simulink model "model_NLMPC_LMPCyawVar"  (R2024b)
settings: Solver=VariableStepAuto  StartTime=0.0  StopTime=25  RelTol=1e-3
undefined symbols (not defined in the file): drone, environment, traj
libraries: sharedtransform x2, mpclib x2, uavutilslib x1
settings Model: Creator=domac  LastModifiedBy=domac

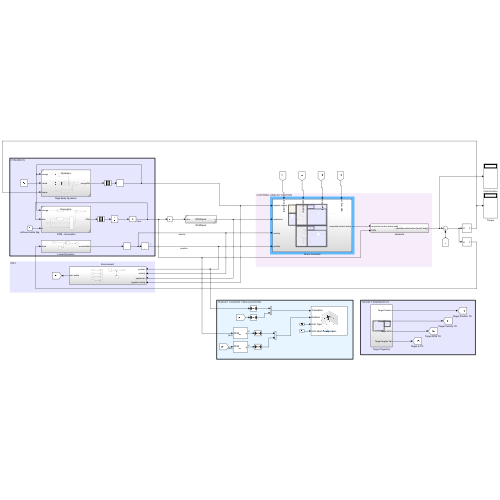
[thumbnail: Simulink's stored preview of the top-level diagram]
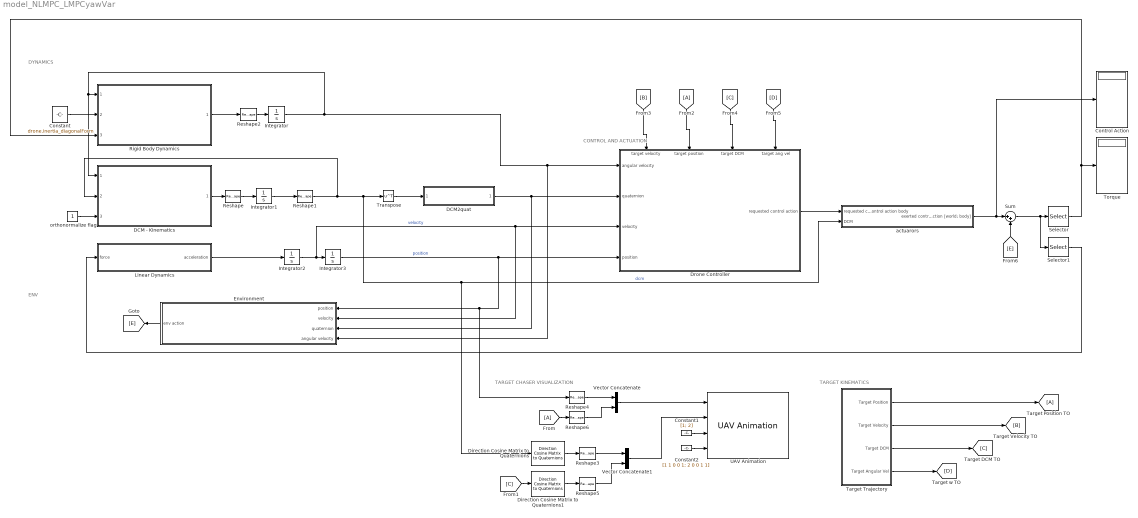
== system model_NLMPC_LMPCyawVar ==
  note: CONTROL AND ACTUATION
  note: DYNAMICS
  note: TARGET KINEMATICS
  note: TARGET CHASER VISUALIZATION
  note: ENV
  " DCM - Kinematics" : Subsystem  ReferencedSubsystem=Kinematics
  Constant : Constant  Value=drone.inertia_diagonalForm  VectorParams1D=off
  Constant1 : Constant  Value=[1; 2]
  Constant2 : Constant  Value=[1 1 0 0 1; 2 0 0 1 1]
  Control Action : Display
  DCM2quat : Subsystem  ReferencedSubsystem=DCM2quat
  Direction Cosine Matrix to Quaternions : sharedtransform/Direction Cosine Matrix  to Quaternions  aMode=0  action=None  tolerance=eps(2)
      settings: LibrarySourceBlock=|
      | aerolibtransform2/Direction Cosine Matrix
      | to Quaternions
  Direction Cosine Matrix to Quaternions1 : sharedtransform/Direction Cosine Matrix  to Quaternions  aMode=0  action=None  tolerance=eps(2)
      settings: LibrarySourceBlock=|
      | aerolibtransform2/Direction Cosine Matrix
      | to Quaternions
  Drone Controller : Subsystem
      settings: PortSchema="{\"entries\":[{\"content\":{\"sides\":[{\"content\":{\"connectorIds\":[\"In1\",\"In2\",\"In3\",\"In4\"]},\"type\":\"ConnectorPlacement.EquallySpacedRectSide\",\"uuid\":\"5cbf5d97-798f-4abe-9063-7d9475aab2f7\"},{\"content\":{\"connectorIds\":[\"Out1\"],\"side\":\"RIGHT\"},\"type\":\"ConnectorPlacement.EquallySpacedRectSide\",\"uuid\":\"8e1c1ff5-210e-451e-9bb4-b2ea9c687a0c\"},{\"content\":{\"connectorIds\":[\"In5\",\"In6\",\"In7\",\"In8\"],\"side\":\"TOP\"},\"type\":\"ConnectorPlacement.EquallySpacedRectSide\",\"uuid\":\"7263c23d-5bc0-464e-848c-51e45572c4cc\"}]},\"type\":\"ConnectorPlacement.EquallySpacedConnector\",\"uuid\":\"7a6c5e6f-7804-4a94-a46d-c2acf2bd8613\"}],\"packageUris\":[\"http://schema.mathworks.com/mf0/Connector/R2020b\"],\"version\":\"1.0\"}"
  Environment : Subsystem
  From : From
  From2 : From
  Integrator : Integrator  InitialCondition=drone.w0
  Integrator1 : Integrator  InitialCondition=[drone.initialDCM(:,1); drone.initialDCM(:,2); drone.initialDCM(:,3)]
  Integrator2 : Integrator  InitialCondition=drone.v0
  Integrator3 : Integrator  InitialCondition=drone.x0
  Linear Dynamics : Subsystem
  Reshape : Reshape  OutputDimensionality=Column vector (2-D)
  Reshape1 : Reshape  OutputDimensionality=Customize  OutputDimensions=[3, 3]
  Reshape2 : Reshape  OutputDimensionality=Column vector (2-D)
  Reshape{3..6} (4 alike) : Reshape  OutputDimensionality=Row vector (2-D)
  Rigid Body Dynamics : Subsystem  ReferencedSubsystem=Dynamics
  Selector : Selector  InputPortWidth=6  IndexOptions=Index vector (dialog)  Indices=[4 5 6]  OutputSizes=1
  Selector1 : Selector  InputPortWidth=6  IndexOptions=Index vector (dialog)  Indices=[1 2 3]  OutputSizes=1
  Sum : Sum  Inputs=|++
  Target Position TO : Goto
  Target Trajectory : Subsystem
  Torque : Display
  Transpose : Math  Operator=transpose
  UAV Animation : uavutilslib/UAV Animation  NumUAV=2  DynamicUAVConfig=on  UAVType=Multirotor  UAVSize=1  UAVColor=[1 0 0]  UAVTrajectoryAlpha=1  InertialZDirection=Up  RotationFormat=Quaternion  DrawMarkers=off  SampleTime=-1
  Vector Concatenate : Concatenate  Mode=Multidimensional array
  Vector Concatenate1 : Concatenate  Mode=Multidimensional array
  actuarors : Subsystem
  orthonormalize flag : Constant
  wires:
  orthonormalize flag/1 -> " DCM - Kinematics"/3
  " DCM - Kinematics"/1 -> Reshape/1
  Integrator1/1 -> Reshape1/1
  Reshape1/1 -> " DCM - Kinematics"/2, Direction Cosine Matrix to Quaternions/1, actuarors/2(DCM), Transpose/1  "dcm"
  Reshape/1 -> Integrator1/1
  Rigid Body Dynamics/1 -> Reshape2/1
  Linear Dynamics/1(acceleration) -> Integrator2/1
  Integrator2/1 -> Drone Controller/3(velocity), Environment/2(velocity), Integrator3/1  "velocity"
  DCM2quat/1 -> Drone Controller/2(quaternion), Environment/3(quaternion)
  Integrator/1 -> " DCM - Kinematics"/1, Rigid Body Dynamics/1, Drone Controller/1(angular velocity), Environment/4(angular velocity)
  Integrator3/1 -> Environment/1(position), Reshape4/1, Drone Controller/4("position ")  "position"
  actuarors/1(exerted control action [world; body]) -> Control Action/1, Sum/1
  Drone Controller/1(requested control action) -> actuarors/1(requested control action body)
  Sum/1 -> Selector/1, Selector1/1
  Selector1/1 -> Linear Dynamics/1(force)
  Target Trajectory/1(Target Position) -> Target Position TO/1
  Selector/1 -> Rigid Body Dynamics/3, Torque/1
  Constant/1 -> Rigid Body Dynamics/2
  Reshape2/1 -> Integrator/1
  Direction Cosine Matrix to Quaternions/1 -> Reshape3/1
  Reshape4/1 -> Vector Concatenate/1
  Vector Concatenate/1 -> UAV Animation/1
  Reshape3/1 -> Vector Concatenate1/1
  Vector Concatenate1/1 -> UAV Animation/2
  Target Trajectory/3(Target DCM) -> [C]
  From/1 -> Reshape6/1
  [C] -> Direction Cosine Matrix to Quaternions1/1
  Direction Cosine Matrix to Quaternions1/1 -> Reshape5/1
  Reshape5/1 -> Vector Concatenate1/2
  Reshape6/1 -> Vector Concatenate/2
  Constant1/1 -> UAV Animation/3
  Constant2/1 -> UAV Animation/4
  Transpose/1 -> DCM2quat/1
  From2/1 -> Drone Controller/6(target position)
  Target Trajectory/2(Target Velocity) -> [B]
  [B] -> Drone Controller/5(target velocity)
  [C] -> Drone Controller/7(target DCM)
  Target Trajectory/4(Target Angular Vel) -> [D]
  [D] -> Drone Controller/8(target ang vel)
  Environment/1(env action) -> [E]
  [E] -> Sum/2

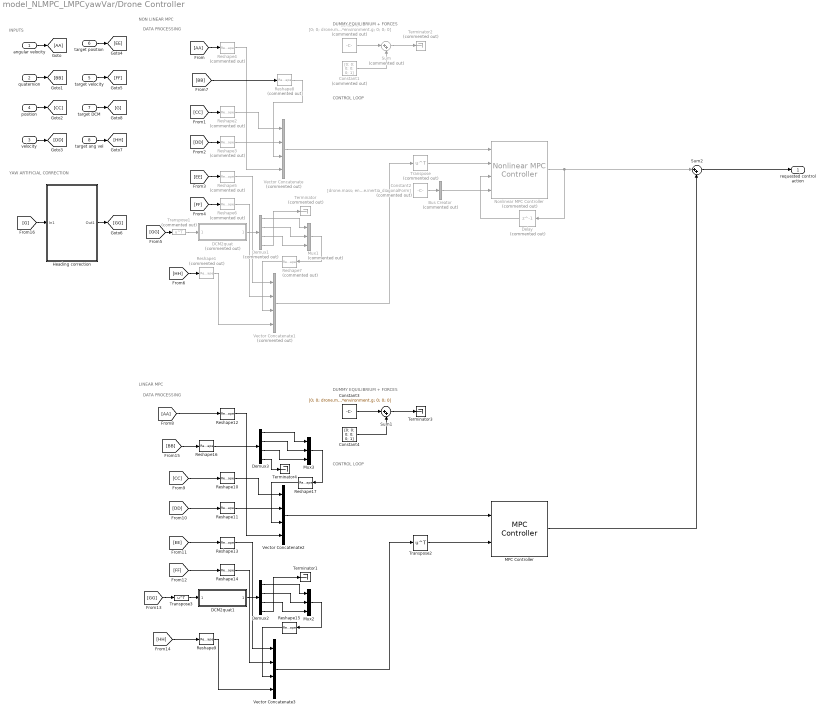
== system model_NLMPC_LMPCyawVar/Drone Controller ==
  note: YAW ARTIFICIAL CORRECTION
  note: NON LINEAR MPC
  note: INPUTS
  note: DATA PROCESSING
  note: CONTROL LOOP
  note: DUMMY EQUILIBRIUM + FORCES
  note: DUMMY EQUILIBRIUM + FORCES
  note: DATA PROCESSING
  note: CONTROL LOOP
  note: LINEAR MPC
  angular velocity : Inport
  quaternion : Inport  Port=2
  velocity : Inport  Port=3
  "position " : Inport  Port=4
  target velocity : Inport  Port=5
  target position : Inport  Port=6
  target DCM : Inport  Port=7
  target ang vel : Inport  Port=8
  Bus Creator : BusCreator  Commented=on  Inputs=1  OutDataTypeStr=Bus: paramsBus  NonVirtualBus=on
      settings: InheritFromInputs=off
  Constant : Constant  Commented=on  Value=[0; 0; drone.m*environment.g; 0; 0; 0]  VectorParams1D=off
  Constant1 : Constant  Commented=on  Value=[0; 0; 0; 0; 0; 1]  VectorParams1D=off
  Constant2 : Constant  Commented=on  Value=[drone.mass; environment.g; drone.inertia_diagonalForm]
  Constant3 : Constant  Value=[0; 0; drone.m*environment.g; 0; 0; 0]  VectorParams1D=off
  Constant4 : Constant  Value=[0; 0; 0; 0; 0; 1]  VectorParams1D=off
  DCM2quat : Subsystem  Commented=on  ReferencedSubsystem=DCM2quat
  DCM2quat1 : Subsystem  ReferencedSubsystem=DCM2quat
  Delay : Delay  Commented=on  DelayLength=1
  Demux1 : Demux  Commented=on
  Demux2 : Demux
  Demux3 : Demux
  Heading correction : Subsystem
  MPC Controller : mpclib/MPC Controller  SCDEnableBlockLinearizationSpecification=on  mpcobj=controllerLin  is_multiple=0  enable_value=0  return_u0=off  updateMPCinCallerWorkspace=on  md_inport=off  mv_inport=off  uref_inport=off  return_cost=off  return_mvseq=off  return_qpstatus=off  return_xseq=off  return_state=off  return_ovseq=off  state_inport=off  umin_inport=off  umax_inport=off  ymin_inport=off  ymax_inport=off  cc_inport=off  ywt_inport=off  uwt_inport=off  duwt_inport=off  rhoeps_inport=off  pm_inport=off  MaximumP=10  HorizonChoice=FixedHorizon  n_ts=0.025  n_p=20  n_mv=4  n_md=0  n_ud=0  n_mo=12  n_uo=0  BlockDataType=double  SampleTimeInherited=off  switch_inport=off
  Mux1 : Mux  Commented=on  Inputs=3
  Mux2 : Mux  Inputs=3
  Mux3 : Mux  Inputs=3
  Nonlinear MPC Controller : mpclib/Nonlinear MPC Controller  Commented=on  nlmpcobj=controller  UseObjectTs=on  UseMEX=off  md_enabled=off  mvtarget_enabled=off  param_enabled=on  cost_enabled=off  mvseq_enabled=off  stateseq_enabled=off  ovseq_enabled=off  slack_enabled=off  status_enabled=off  ov_min=off  ov_max=off  mv_min=off  mv_max=off  mvrate_min=off  mvrate_max=off  state_min=off  state_max=off  ov_weight=off  mv_weight=off  mvrate_weight=off  ecr_weight=off  nlp_initialize=off
  Reshape{1..8} (8 alike) : Reshape  Commented=on  OutputDimensionality=Column vector (2-D)
  Reshape{9..17} (9 alike) : Reshape  OutputDimensionality=Column vector (2-D)
  Sum : Sum  Commented=on  Inputs=|++
  Sum1 : Sum  Inputs=|++
  Sum2 : Sum  Inputs=|++
  Terminator : Terminator  Commented=on
  Terminator1 : Terminator
  Terminator2 : Terminator  Commented=on
  Terminator3 : Terminator
  Terminator4 : Terminator
  Transpose : Math  Commented=on  Operator=transpose
  Transpose1 : Math  Commented=on  Operator=transpose
  Transpose2 : Math  Operator=transpose
  Transpose3 : Math  Operator=transpose
  Vector Concatenate : Concatenate  Commented=on  NumInputs=4
  Vector Concatenate1 : Concatenate  Commented=on  NumInputs=4
  Vector Concatenate2 : Concatenate  NumInputs=4
  Vector Concatenate3 : Concatenate  NumInputs=4
  requested control action : Outport
  wires:
  Constant/1 -> Sum/1
  Constant1/1 -> Sum/2
  Nonlinear MPC Controller/1 -> Sum2/1, Delay/1
  Delay/1 -> Nonlinear MPC Controller/3
  Reshape3/1 -> Vector Concatenate/2
  Reshape2/1 -> Vector Concatenate/1
  Reshape8/1 -> Vector Concatenate/3
  Vector Concatenate/1 -> Nonlinear MPC Controller/1
  DCM2quat/1 -> Demux1/1
  Mux1/1 -> Reshape7/1
  Reshape5/1 -> Vector Concatenate1/1
  Reshape6/1 -> Vector Concatenate1/2
  Vector Concatenate1/1 -> Transpose/1
  Reshape1/1 -> Vector Concatenate1/4
  Reshape7/1 -> Vector Concatenate1/3
  Sum/1 -> Terminator2/1
  Constant2/1 -> Bus Creator/1
  Bus Creator/1 -> Nonlinear MPC Controller/4
  Reshape4/1 -> Vector Concatenate/4
  Transpose/1 -> Nonlinear MPC Controller/2
  Transpose1/1 -> DCM2quat/1
  Demux1/4 -> Terminator/1
  Demux1/2 -> Mux1/2
  Demux1/1 -> Mux1/1
  Demux1/3 -> Mux1/3
  Transpose2/1 -> MPC Controller/2
  Vector Concatenate2/1 -> MPC Controller/1
  [FF] -> Reshape14/1
  Demux2/2 -> Mux2/2
  Reshape10/1 -> Vector Concatenate2/1
  Reshape12/1 -> Vector Concatenate2/4
  Reshape15/1 -> Vector Concatenate3/3
  Constant4/1 -> Sum1/2
  [HH] -> Reshape9/1
  Vector Concatenate3/1 -> Transpose2/1
  Reshape9/1 -> Vector Concatenate3/4
  Constant3/1 -> Sum1/1
  Demux2/1 -> Mux2/1
  [CC] -> Reshape10/1
  DCM2quat1/1 -> Demux2/1
  [BB] -> Reshape16/1
  Reshape11/1 -> Vector Concatenate2/2
  Reshape17/1 -> Vector Concatenate2/3
  [DD] -> Reshape11/1
  Reshape14/1 -> Vector Concatenate3/2
  Mux3/1 -> Reshape17/1
  [EE] -> Reshape13/1
  Mux2/1 -> Reshape15/1
  Reshape16/1 -> Demux3/1
  Demux3/1 -> Mux3/1
  Sum1/1 -> Terminator3/1
  [AA] -> Reshape12/1
  Demux3/4 -> Terminator4/1
  Demux3/3 -> Mux3/3
  Demux2/4 -> Terminator1/1
  Transpose3/1 -> DCM2quat1/1
  Demux3/2 -> Mux3/2
  Reshape13/1 -> Vector Concatenate3/1
  MPC Controller/1 -> Sum2/2
  Demux2/3 -> Mux2/3
  Sum2/1 -> requested control action/1
  angular velocity/1 -> [AA]
  quaternion/1 -> [BB]
  velocity/1 -> [DD]
  "position "/1 -> [CC]
  target position/1 -> [EE]
  target velocity/1 -> [FF]
  target ang vel/1 -> [HH]
  [AA] -> Reshape4/1
  [CC] -> Reshape2/1
  [DD] -> Reshape3/1
  [EE] -> Reshape5/1
  [FF] -> Reshape6/1
  [GG] -> Transpose1/1
  [HH] -> Reshape1/1
  [GG] -> Transpose3/1
  [BB] -> Reshape8/1
  target DCM/1 -> [G]
  [G] -> Heading correction/1(In1)
  Heading correction/1(Out1) -> [GG]

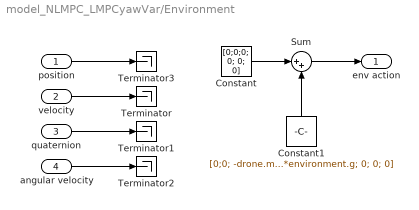
== system model_NLMPC_LMPCyawVar/Environment ==
  position : Inport
  velocity : Inport  Port=2
  quaternion : Inport  Port=3
  angular velocity : Inport  Port=4
  Constant : Constant  Value=[0;0;0; 0; 0; 0]
  Constant1 : Constant  Value=[0;0; -drone.m*environment.g; 0; 0; 0]
  Sum : Sum  Inputs=|++
  Terminator{,1..3} (4 alike) : Terminator
  env action : Outport
  wires:
  velocity/1 -> Terminator/1
  angular velocity/1 -> Terminator2/1
  quaternion/1 -> Terminator1/1
  position/1 -> Terminator3/1
  Constant/1 -> Sum/1
  Constant1/1 -> Sum/2
  Sum/1 -> env action/1

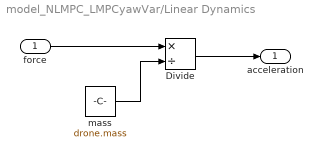
== system model_NLMPC_LMPCyawVar/Linear Dynamics ==
  force : Inport
  Divide : Product  Inputs=*/
  mass : Constant  Value=drone.mass
  acceleration : Outport
  wires:
  force/1 -> Divide/1
  mass/1 -> Divide/2
  Divide/1 -> acceleration/1

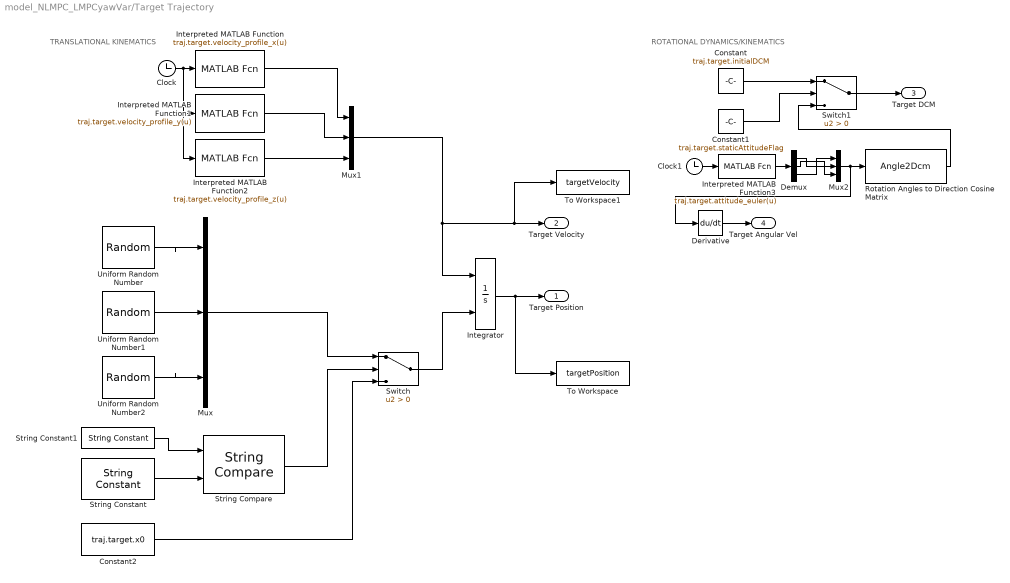
== system model_NLMPC_LMPCyawVar/Target Trajectory ==
  note: ROTATIONAL
      | DYNAMICS/KINEMATICS
  note: TRANSLATIONAL
      | KINEMATICS
  Clock : Clock
  Clock1 : Clock
  Constant : Constant  Value=traj.target.initialDCM  VectorParams1D=off
  Constant1 : Constant  Value=traj.target.staticAttitudeFlag
  Constant2 : Constant  Value=traj.target.x0
  Demux : Demux  Outputs=3
  Derivative : Derivative
  Integrator : Integrator  InitialConditionSource=external
  Interpreted MATLAB Function : MATLABFcn  MATLABFcn=traj.target.velocity_profile_x(u)  OutputDimensions=1
  Interpreted MATLAB Function1 : MATLABFcn  MATLABFcn=traj.target.velocity_profile_y(u)  OutputDimensions=1
  Interpreted MATLAB Function2 : MATLABFcn  MATLABFcn=traj.target.velocity_profile_z(u)  OutputDimensions=1
  Interpreted MATLAB Function3 : MATLABFcn  MATLABFcn=traj.target.attitude_euler(u)
  Mux : Mux  Inputs=3
  Mux1 : Mux  Inputs=3
  Mux2 : Mux  Inputs=3
  Rotation Angles to Direction Cosine Matrix : Angle2Dcm
      settings: AttributesFormatString=Rotation Order: %<rotationOrder>
  String Compare : StringCompare
  String Constant : StringConstant  String="\"random\""
  String Constant1 : StringConstant  String=traj.target.x0Type
  Switch : Switch  Criteria=u2 > Threshold  SaturateOnIntegerOverflow=off  InputSameDT=off
  Switch1 : Switch  Criteria=u2 > Threshold  SaturateOnIntegerOverflow=off  InputSameDT=off
  To Workspace : ToWorkspace  VariableName=targetPosition  SaveFormat=Timeseries  SampleTime=-1
  To Workspace1 : ToWorkspace  VariableName=targetVelocity  SaveFormat=Timeseries  SampleTime=-1
  Uniform Random Number : UniformRandomNumber  Minimum=-10  Maximum=10  SampleTime=0.1
  Uniform Random Number1 : UniformRandomNumber  Minimum=-10  Maximum=10  SampleTime=0.1
  Uniform Random Number2 : UniformRandomNumber  Minimum=-10  Maximum=10  SampleTime=0.1
  Target Position : Outport
  Target Velocity : Outport  Port=2
  Target DCM : Outport  Port=3
  Target Angular Vel : Outport  Port=4
  wires:
  Uniform Random Number1/1 -> Mux/2
  Uniform Random Number/1 -> Mux/1
  Uniform Random Number2/1 -> Mux/3
  Mux/1 -> Switch/1
  Clock/1 -> Interpreted MATLAB Function2/1, Interpreted MATLAB Function1/1, Interpreted MATLAB Function/1
  Mux1/1 -> Integrator/1, To Workspace1/1, Target Velocity/1
  String Constant/1 -> String Compare/2
  String Constant1/1 -> String Compare/1
  Switch/1 -> Integrator/2
  String Compare/1 -> Switch/2
  Constant2/1 -> Switch/3
  Integrator/1 -> To Workspace/1, Target Position/1
  Interpreted MATLAB Function/1 -> Mux1/1
  Interpreted MATLAB Function1/1 -> Mux1/2
  Interpreted MATLAB Function2/1 -> Mux1/3
  Constant/1 -> Switch1/1
  Constant1/1 -> Switch1/2
  Clock1/1 -> Interpreted MATLAB Function3/1
  Switch1/1 -> Target DCM/1
  Rotation Angles to Direction Cosine Matrix/1 -> Switch1/3
  Interpreted MATLAB Function3/1 -> Demux/1
  Mux2/1 -> Derivative/1, Rotation Angles to Direction Cosine Matrix/1
  Demux/3 -> Mux2/1
  Demux/1 -> Mux2/3
  Demux/2 -> Mux2/2
  Derivative/1 -> Target Angular Vel/1

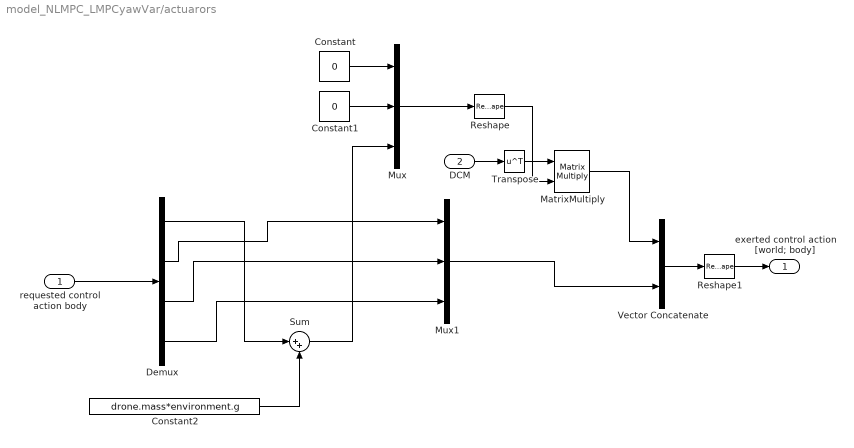
== system model_NLMPC_LMPCyawVar/actuarors ==
  requested control action body : Inport
  DCM : Inport  Port=2
  Constant : Constant  Value=0
  Constant1 : Constant  Value=0
  Constant2 : Constant  Value=drone.mass*environment.g
  Demux : Demux
  MatrixMultiply : Product  Multiplication=Matrix(*)
  Mux : Mux  Inputs=3
  Mux1 : Mux  Inputs=3
  Reshape : Reshape  OutputDimensionality=Column vector (2-D)
  Reshape1 : Reshape  OutputDimensionality=Column vector (2-D)
  Sum : Sum  Inputs=|++
  Transpose : Math  Operator=transpose
  Vector Concatenate : Concatenate
  exerted control action [world; body] : Outport
  wires:
  Constant/1 -> Mux/1
  Constant1/1 -> Mux/2
  requested control action body/1 -> Demux/1
  DCM/1 -> Transpose/1
  Mux/1 -> Reshape/1
  Reshape/1 -> MatrixMultiply/2
  MatrixMultiply/1 -> Vector Concatenate/1
  Mux1/1 -> Vector Concatenate/2
  Vector Concatenate/1 -> Reshape1/1
  Reshape1/1 -> exerted control action [world; body]/1
  Sum/1 -> Mux/3
  Constant2/1 -> Sum/2
  Demux/1 -> Sum/1
  Demux/4 -> Mux1/3
  Demux/3 -> Mux1/2
  Demux/2 -> Mux1/1
  Transpose/1 -> MatrixMultiply/1

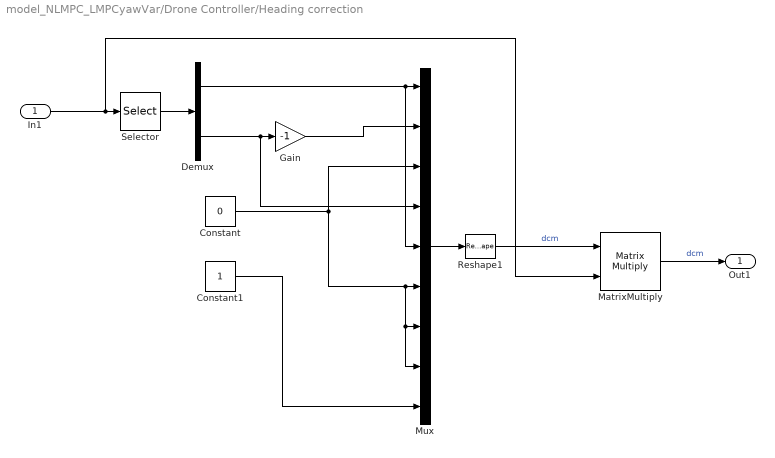
== system model_NLMPC_LMPCyawVar/Drone Controller/Heading correction ==
  In1 : Inport
  Constant : Constant  Value=0
  Constant1 : Constant
  Demux : Demux  Outputs=2
  Gain : Gain  Gain=-1
  MatrixMultiply : Product  Multiplication=Matrix(*)
  Mux : Mux  Inputs=9
  Reshape1 : Reshape  OutputDimensionality=Customize  OutputDimensions=[3, 3]
  Selector : Selector  NumberOfDimensions=2  InputPortWidth=3  IndexOptions=Index vector (dialog),Index vector (dialog)  Indices=1,[1 2]  OutputSizes=1,1
  Out1 : Outport
  wires:
  MatrixMultiply/1 -> Out1/1  "dcm"
  In1/1 -> MatrixMultiply/2, Selector/1
  Selector/1 -> Demux/1
  Demux/1 -> Mux/5, Mux/1
  Demux/2 -> Mux/4, Gain/1
  Gain/1 -> Mux/2
  Constant/1 -> Mux/8, Mux/7, Mux/6, Mux/3
  Constant1/1 -> Mux/9
  Mux/1 -> Reshape1/1
  Reshape1/1 -> MatrixMultiply/1  "dcm"
